simulink model "HFB_Comb4_Comb4"  (R2022b)
settings: Solver=FixedStepDiscrete  StartTime=0.0  StopTime=0.01  RelTol=1e-3
libraries: dspsigops x10, dspsrcs4 x1
settings Model: Creator=ASAA  LastModifiedBy=ASAA

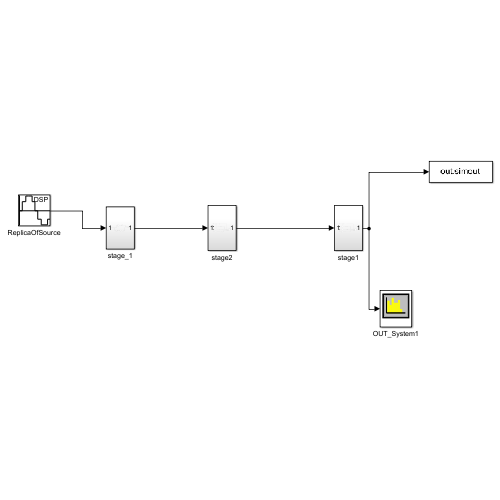
[thumbnail: Simulink's stored preview of the top-level diagram]
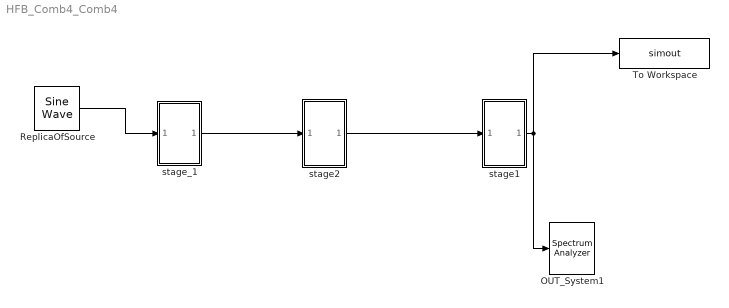
== system HFB_Comb4_Comb4 ==
  OUT_System1 : SpectrumAnalyzer
  ReplicaOfSource : dspsrcs4/Sine Wave  Amplitude=0.6  Frequency=100e3  Phase=0  SampleMode=Discrete  OutComplex=Real  CompMethod=Trigonometric fcn  TableSize=Speed  SampleTime=1/3.125e6  SamplesPerFrame=1  ResetState=Restart at time zero  OutputFrames=off  dataType=double  wordLen=16  udDataType=sfix(16)  fracBitsMode=Best precision  numFracBits=15  OutDataTypeStr=double  LastOutDataTypeStr=double
  To Workspace : ToWorkspace  VariableName=simout  SaveFormat=Timeseries  SampleTime=-1
  stage1 : Subsystem
  stage2 : Subsystem
  stage_1 : Subsystem
  wires:
  stage2/1(Out1) -> stage1/1(In1)
  stage_1/1(Out1) -> stage2/1(In1)
  ReplicaOfSource/1 -> stage_1/1(In1)
  stage1/1(Out1) -> OUT_System1/1, To Workspace/1

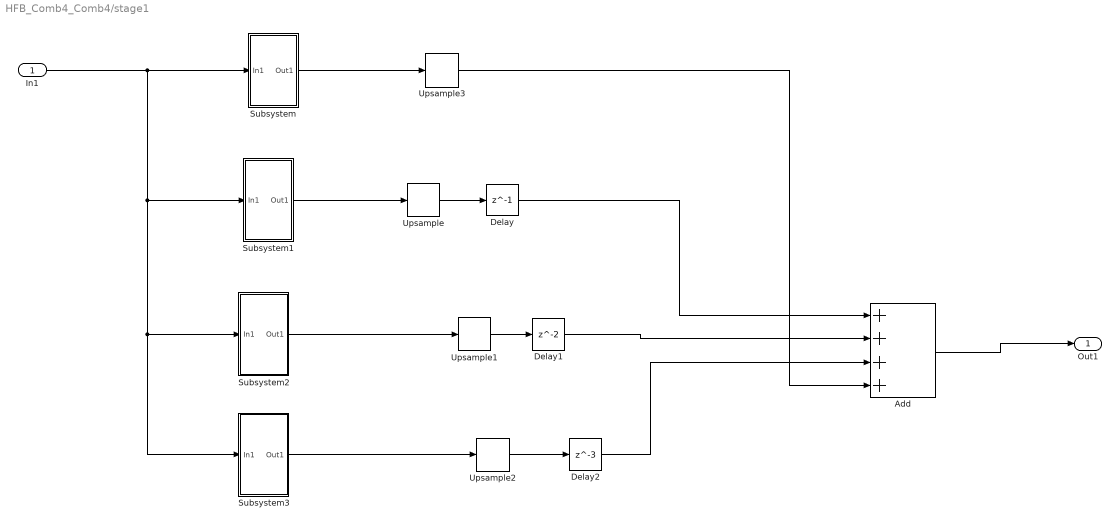
== system HFB_Comb4_Comb4/stage1 ==
  In1 : Inport
  Add : Sum  Inputs=++++
  Delay : Delay  DelayLength=1  InitialCondition=0
  Delay1 : Delay  InitialCondition=0
  Delay2 : Delay  DelayLength=3  InitialCondition=0
  Subsystem : Subsystem
  Subsystem1 : Subsystem
  Subsystem2 : Subsystem
  Subsystem3 : Subsystem
  Upsample{,1..3} (4 alike) : dspsigops/Upsample  N=4  phase=0  RateOptions=Allow multirate processing  ic=0  mode=Unused parameter value
  Out1 : Outport
  wires:
  In1/1 -> Subsystem3/1(In1), Subsystem2/1(In1), Subsystem1/1(In1), Subsystem/1(In1)
  Add/1 -> Out1/1
  Upsample3/1 -> Add/4
  Subsystem/1(Out1) -> Upsample3/1
  Upsample/1 -> Delay/1
  Upsample1/1 -> Delay1/1
  Upsample2/1 -> Delay2/1
  Subsystem1/1(Out1) -> Upsample/1
  Subsystem2/1(Out1) -> Upsample1/1
  Subsystem3/1(Out1) -> Upsample2/1
  Delay/1 -> Add/1
  Delay1/1 -> Add/2
  Delay2/1 -> Add/3

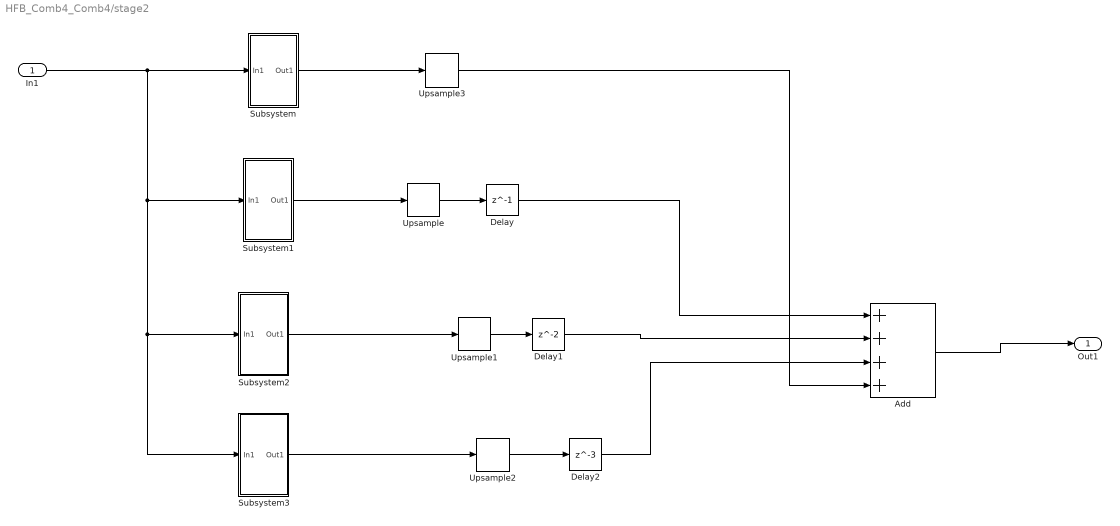
== system HFB_Comb4_Comb4/stage2 ==
  In1 : Inport
  Add : Sum  Inputs=++++
  Delay : Delay  DelayLength=1  InitialCondition=0
  Delay1 : Delay  InitialCondition=0
  Delay2 : Delay  DelayLength=3  InitialCondition=0
  Subsystem : Subsystem
  Subsystem1 : Subsystem
  Subsystem2 : Subsystem
  Subsystem3 : Subsystem
  Upsample{,1..3} (4 alike) : dspsigops/Upsample  N=4  phase=0  RateOptions=Allow multirate processing  ic=0  mode=Unused parameter value
  Out1 : Outport
  wires:
  In1/1 -> Subsystem3/1(In1), Subsystem2/1(In1), Subsystem1/1(In1), Subsystem/1(In1)
  Add/1 -> Out1/1
  Upsample3/1 -> Add/4
  Subsystem/1(Out1) -> Upsample3/1
  Upsample/1 -> Delay/1
  Upsample1/1 -> Delay1/1
  Upsample2/1 -> Delay2/1
  Subsystem1/1(Out1) -> Upsample/1
  Subsystem2/1(Out1) -> Upsample1/1
  Subsystem3/1(Out1) -> Upsample2/1
  Delay/1 -> Add/1
  Delay1/1 -> Add/2
  Delay2/1 -> Add/3

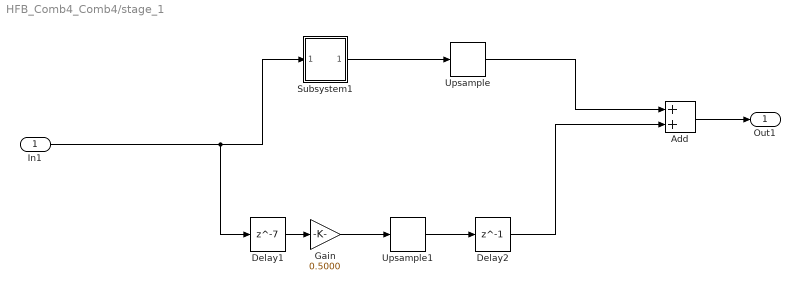
== system HFB_Comb4_Comb4/stage_1 ==
  In1 : Inport
  Add : Sum
  Delay1 : Delay  DelayLength=7  InitialCondition=0
  Delay2 : Delay  DelayLength=1  InitialCondition=0
  Gain : Gain  Gain=0.5000
  Subsystem1 : Subsystem
  Upsample : dspsigops/Upsample  N=2  phase=0  RateOptions=Allow multirate processing  ic=0  mode=Unused parameter value
  Upsample1 : dspsigops/Upsample  N=2  phase=0  RateOptions=Allow multirate processing  ic=0  mode=Unused parameter value
  Out1 : Outport
  wires:
  Add/1 -> Out1/1
  Delay2/1 -> Add/2
  Upsample1/1 -> Delay2/1
  In1/1 -> Delay1/1, Subsystem1/1(In1)
  Delay1/1 -> Gain/1
  Subsystem1/1(Out2) -> Upsample/1
  Upsample/1 -> Add/1
  Gain/1 -> Upsample1/1

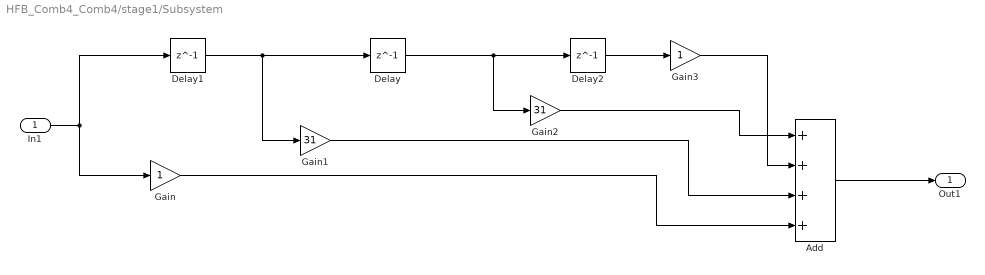
== system HFB_Comb4_Comb4/stage1/Subsystem ==
  In1 : Inport
  Add : Sum  Inputs=++++
  Delay : Delay  DelayLength=1  InitialCondition=0
  Delay1 : Delay  DelayLength=1  InitialCondition=0
  Delay2 : Delay  DelayLength=1  InitialCondition=0
  Gain : Gain
  Gain1 : Gain  Gain=31
  Gain2 : Gain  Gain=31
  Gain3 : Gain
  Out1 : Outport
  wires:
  Delay1/1 -> Gain1/1, Delay/1
  Gain/1 -> Add/4
  In1/1 -> Gain/1, Delay1/1
  Gain2/1 -> Add/1
  Gain1/1 -> Add/3
  Delay/1 -> Delay2/1, Gain2/1
  Add/1 -> Out1/1
  Delay2/1 -> Gain3/1
  Gain3/1 -> Add/2

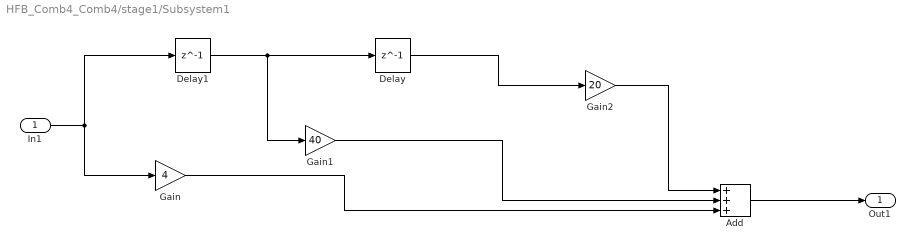
== system HFB_Comb4_Comb4/stage1/Subsystem1 ==
  In1 : Inport
  Add : Sum  Inputs=+++
  Delay : Delay  DelayLength=1  InitialCondition=0
  Delay1 : Delay  DelayLength=1  InitialCondition=0
  Gain : Gain  Gain=4
  Gain1 : Gain  Gain=40
  Gain2 : Gain  Gain=20
  Out1 : Outport
  wires:
  Delay1/1 -> Gain1/1, Delay/1
  Delay/1 -> Gain2/1
  Gain1/1 -> Add/2
  Gain/1 -> Add/3
  Add/1 -> Out1/1
  In1/1 -> Gain/1, Delay1/1
  Gain2/1 -> Add/1

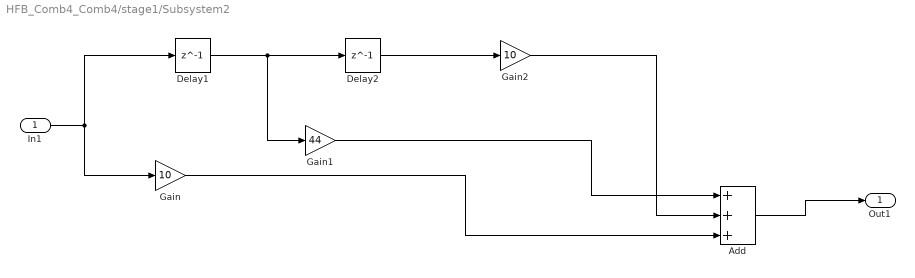
== system HFB_Comb4_Comb4/stage1/Subsystem2 ==
  In1 : Inport
  Add : Sum  Inputs=+++
  Delay1 : Delay  DelayLength=1  InitialCondition=0
  Delay2 : Delay  DelayLength=1  InitialCondition=0
  Gain : Gain  Gain=10
  Gain1 : Gain  Gain=44
  Gain2 : Gain  Gain=10
  Out1 : Outport
  wires:
  Delay1/1 -> Delay2/1, Gain1/1
  Gain1/1 -> Add/1
  Gain/1 -> Add/3
  Add/1 -> Out1/1
  In1/1 -> Gain/1, Delay1/1
  Delay2/1 -> Gain2/1
  Gain2/1 -> Add/2

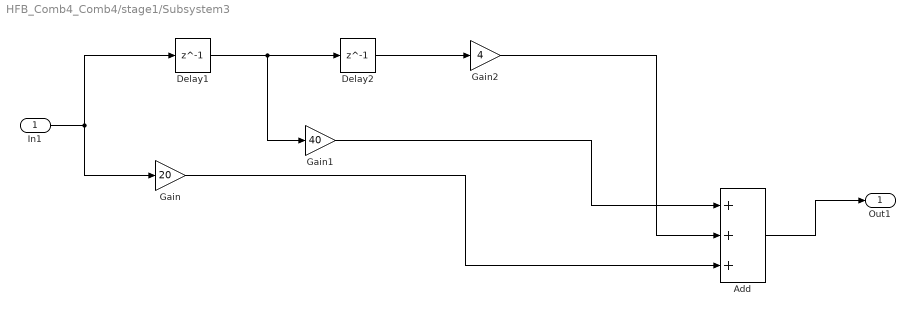
== system HFB_Comb4_Comb4/stage1/Subsystem3 ==
  In1 : Inport
  Add : Sum  Inputs=+++
  Delay1 : Delay  DelayLength=1  InitialCondition=0
  Delay2 : Delay  DelayLength=1  InitialCondition=0
  Gain : Gain  Gain=20
  Gain1 : Gain  Gain=40
  Gain2 : Gain  Gain=4
  Out1 : Outport
  wires:
  Delay1/1 -> Delay2/1, Gain1/1
  Gain1/1 -> Add/1
  Gain/1 -> Add/3
  Add/1 -> Out1/1
  In1/1 -> Gain/1, Delay1/1
  Gain2/1 -> Add/2
  Delay2/1 -> Gain2/1

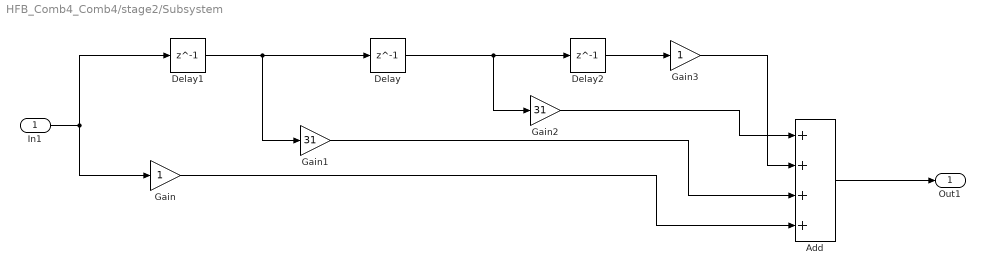
== system HFB_Comb4_Comb4/stage2/Subsystem ==
  In1 : Inport
  Add : Sum  Inputs=++++
  Delay : Delay  DelayLength=1  InitialCondition=0
  Delay1 : Delay  DelayLength=1  InitialCondition=0
  Delay2 : Delay  DelayLength=1  InitialCondition=0
  Gain : Gain
  Gain1 : Gain  Gain=31
  Gain2 : Gain  Gain=31
  Gain3 : Gain
  Out1 : Outport
  wires:
  Delay1/1 -> Gain1/1, Delay/1
  Gain/1 -> Add/4
  In1/1 -> Gain/1, Delay1/1
  Gain2/1 -> Add/1
  Gain1/1 -> Add/3
  Delay/1 -> Delay2/1, Gain2/1
  Add/1 -> Out1/1
  Delay2/1 -> Gain3/1
  Gain3/1 -> Add/2

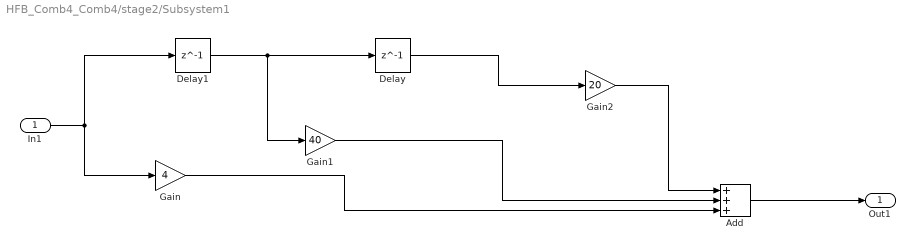
== system HFB_Comb4_Comb4/stage2/Subsystem1 ==
  In1 : Inport
  Add : Sum  Inputs=+++
  Delay : Delay  DelayLength=1  InitialCondition=0
  Delay1 : Delay  DelayLength=1  InitialCondition=0
  Gain : Gain  Gain=4
  Gain1 : Gain  Gain=40
  Gain2 : Gain  Gain=20
  Out1 : Outport
  wires:
  Delay1/1 -> Gain1/1, Delay/1
  Delay/1 -> Gain2/1
  Gain1/1 -> Add/2
  Gain/1 -> Add/3
  Add/1 -> Out1/1
  In1/1 -> Gain/1, Delay1/1
  Gain2/1 -> Add/1

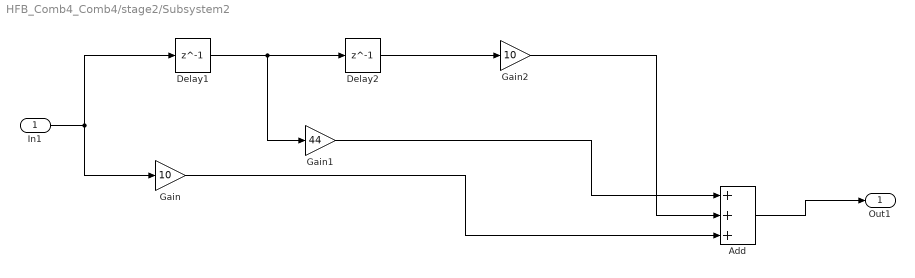
== system HFB_Comb4_Comb4/stage2/Subsystem2 ==
  In1 : Inport
  Add : Sum  Inputs=+++
  Delay1 : Delay  DelayLength=1  InitialCondition=0
  Delay2 : Delay  DelayLength=1  InitialCondition=0
  Gain : Gain  Gain=10
  Gain1 : Gain  Gain=44
  Gain2 : Gain  Gain=10
  Out1 : Outport
  wires:
  Delay1/1 -> Delay2/1, Gain1/1
  Gain1/1 -> Add/1
  Gain/1 -> Add/3
  Add/1 -> Out1/1
  In1/1 -> Gain/1, Delay1/1
  Delay2/1 -> Gain2/1
  Gain2/1 -> Add/2

== system HFB_Comb4_Comb4/stage2/Subsystem3 ==
  In1 : Inport
  Add : Sum  Inputs=+++
  Delay1 : Delay  DelayLength=1  InitialCondition=0
  Delay2 : Delay  DelayLength=1  InitialCondition=0
  Gain : Gain  Gain=20
  Gain1 : Gain  Gain=40
  Gain2 : Gain  Gain=4
  Out1 : Outport
  wires:
  Delay1/1 -> Delay2/1, Gain1/1
  Gain1/1 -> Add/1
  Gain/1 -> Add/3
  Add/1 -> Out1/1
  In1/1 -> Gain/1, Delay1/1
  Gain2/1 -> Add/2
  Delay2/1 -> Gain2/1

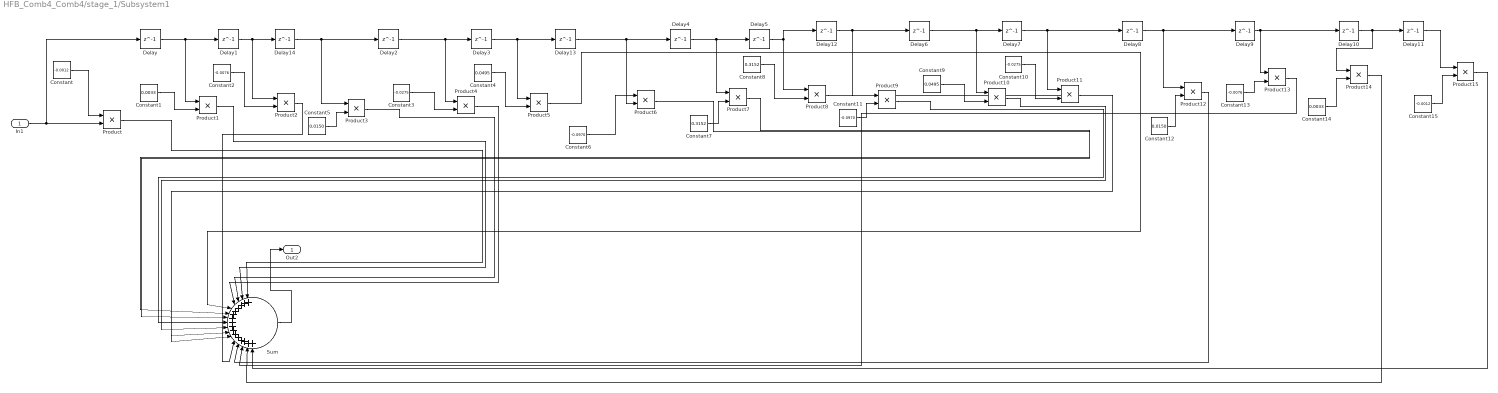
== system HFB_Comb4_Comb4/stage_1/Subsystem1 ==
  In1 : Inport
  Constant : Constant  Value=-0.0012
  Constant1 : Constant  Value=0.0033
  Constant10 : Constant  Value=-0.0275
  Constant11 : Constant  Value=-0.0970
  Constant12 : Constant  Value=0.0150
  Constant13 : Constant  Value=-0.0076
  Constant14 : Constant  Value=0.0033
  Constant15 : Constant  Value=-0.0012
  Constant2 : Constant  Value=-0.0076
  Constant3 : Constant  Value=-0.0275
  Constant4 : Constant  Value=0.0495
  Constant5 : Constant  Value=0.0150
  Constant6 : Constant  Value=-0.0970
  Constant7 : Constant  Value=0.3152
  Constant8 : Constant  Value=0.3152
  Constant9 : Constant  Value=0.0495
  Delay{,1..14} (15 alike) : Delay  DelayLength=1  InitialCondition=0
  Product{,1..15} (16 alike) : Product
  Sum : Sum  Inputs=|++++++++++++++++
  Out2 : Outport
  wires:
  Constant1/1 -> Product1/2
  Delay2/1 -> Delay3/1, Product4/1
  Constant10/1 -> Product11/2
  Constant9/1 -> Product10/2
  Delay/1 -> Delay1/1, Product1/1
  Delay4/1 -> Delay5/1, Product7/1
  Constant3/1 -> Product4/2
  Product8/1 -> Sum/11
  Product6/1 -> Sum/6
  Delay1/1 -> Product2/1, Delay14/1
  Delay5/1 -> Delay12/1, Product8/1
  Constant8/1 -> Product8/2
  In1/1 -> Delay/1, Product/2
  Delay6/1 -> Delay7/1, Product10/1
  Constant/1 -> Product/1
  Constant11/1 -> Product9/2
  Product10/1 -> Sum/9
  Delay7/1 -> Delay8/1, Product11/1
  Product9/1 -> Sum/8
  Delay3/1 -> Product5/1, Delay13/1
  Constant4/1 -> Product5/2
  Product3/1 -> Sum/3
  Product5/1 -> Sum/5
  Constant2/1 -> Product2/2
  Constant5/1 -> Product3/2
  Constant7/1 -> Product7/2
  Product11/1 -> Sum/10
  Constant6/1 -> Product6/1
  Product/1 -> Sum/1
  Product1/1 -> Sum/2
  Product7/1 -> Sum/7
  Product4/1 -> Sum/4
  Sum/1 -> Out2/1
  Product2/1 -> Sum/12
  Constant12/1 -> Product12/2
  Delay8/1 -> Product12/1, Delay9/1
  Constant13/1 -> Product13/2
  Delay9/1 -> Delay10/1, Product13/1
  Constant14/1 -> Product14/2
  Delay10/1 -> Delay11/1, Product14/1
  Delay11/1 -> Product15/1
  Constant15/1 -> Product15/2
  Product12/1 -> Sum/13
  Product13/1 -> Sum/14
  Product14/1 -> Sum/15
  Product15/1 -> Sum/16
  Delay12/1 -> Delay6/1, Product9/1
  Delay13/1 -> Delay4/1, Product6/2
  Delay14/1 -> Delay2/1, Product3/1
